simulink model "fir_import_compare"  (R2026a)
settings: Solver=FixedStepDiscrete  StopTime=300  FixedStep=1
model workspace (MAT data in the model file):
  b = [0.125 0.375 0.375 0.125]
  f_noise = 0.4
  f_sig = 0.01
settings Model: Creator=KoayXianCong  LastModifiedBy=KoayXianCong

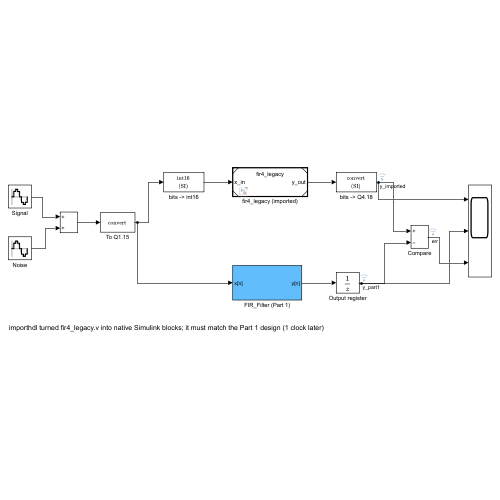
[thumbnail: Simulink's stored preview of the top-level diagram]
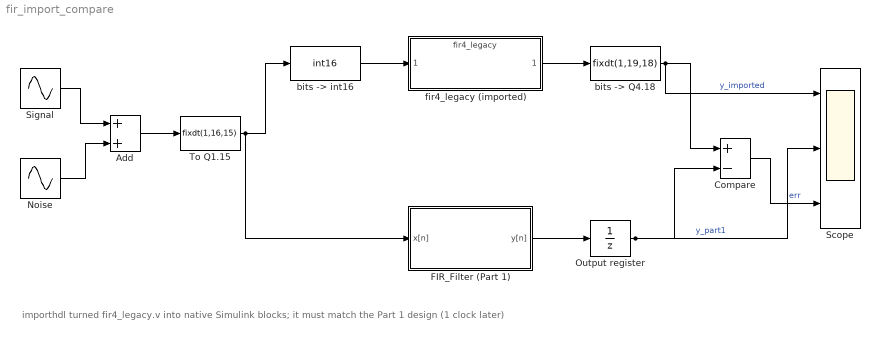
== system fir_import_compare ==
  note: importhdl turned fir4_legacy.v into native Simulink blocks; it must match the Part 1 design (1 clock later)
  Add : Sum
  Compare : Sum  Inputs=+-
  FIR_Filter (Part 1) : Subsystem
  Noise : Sin  Amplitude=0.4  Frequency=2*pi*f_noise  SampleTime=1
  Output register : UnitDelay  SampleTime=-1
  Scope : Scope  NumInputPorts=3
      settings: TimeSpan=300
  Signal : Sin  Amplitude=0.5  Frequency=2*pi*f_sig  SampleTime=1
  To Q1.15 : DataTypeConversion  OutDataTypeStr=fixdt(1,16,15)  RndMeth=Nearest
  "bits -> Q4.18" : DataTypeConversion  OutDataTypeStr=fixdt(1,19,18)  ConvertRealWorld=Stored Integer (SI)  SaturateOnIntegerOverflow=off  RndMeth=Floor
  "bits -> int16" : DataTypeConversion  OutDataTypeStr=int16  ConvertRealWorld=Stored Integer (SI)  SaturateOnIntegerOverflow=off  RndMeth=Floor
  fir4_legacy (imported) : ModelReference  ModelNameDialog=fir4_legacy  SimulationMode=Normal  ModelReferenceVersion=1.1
  wires:
  Signal/1 -> Add/1
  Noise/1 -> Add/2
  Add/1 -> To Q1.15/1
  To Q1.15/1 -> "bits -> int16"/1, FIR_Filter (Part 1)/1(x[n])
  "bits -> int16"/1 -> fir4_legacy (imported)/1
  fir4_legacy (imported)/1 -> "bits -> Q4.18"/1
  FIR_Filter (Part 1)/1(y[n]) -> Output register/1
  "bits -> Q4.18"/1 -> Compare/1, Scope/1  "y_imported"
  Output register/1 -> Compare/2, Scope/2  "y_part1"
  Compare/1 -> Scope/3  "err"

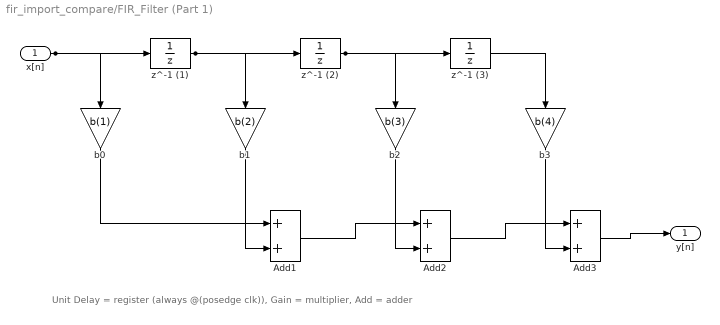
== system fir_import_compare/FIR_Filter (Part 1) ==
  note: Unit Delay = register (always @(posedge clk)), Gain = multiplier, Add = adder
  x[n] : Inport
  Add1 : Sum  OutDataTypeStr=fixdt(1,19,18)
  Add2 : Sum  OutDataTypeStr=fixdt(1,19,18)
  Add3 : Sum  OutDataTypeStr=fixdt(1,19,18)
  b0 : Gain  Gain=b(1)  ParamDataTypeStr=fixdt(1,16,15)  OutDataTypeStr=fixdt(1,19,18)
  b1 : Gain  Gain=b(2)  ParamDataTypeStr=fixdt(1,16,15)  OutDataTypeStr=fixdt(1,19,18)
  b2 : Gain  Gain=b(3)  ParamDataTypeStr=fixdt(1,16,15)  OutDataTypeStr=fixdt(1,19,18)
  b3 : Gain  Gain=b(4)  ParamDataTypeStr=fixdt(1,16,15)  OutDataTypeStr=fixdt(1,19,18)
  z^-1 (1) : UnitDelay  SampleTime=-1
  z^-1 (2) : UnitDelay  SampleTime=-1
  z^-1 (3) : UnitDelay  SampleTime=-1
  y[n] : Outport
  wires:
  Add3/1 -> y[n]/1
  b3/1 -> Add3/2
  Add2/1 -> Add3/1
  b2/1 -> Add2/2
  Add1/1 -> Add2/1
  b1/1 -> Add1/2
  b0/1 -> Add1/1
  z^-1 (3)/1 -> b3/1
  z^-1 (2)/1 -> b2/1, z^-1 (3)/1
  z^-1 (1)/1 -> b1/1, z^-1 (2)/1
  x[n]/1 -> b0/1, z^-1 (1)/1
